simulink model "inverted_pendulum_simulink"  (R2025a)
settings: Solver=ode45  StartTime=0.0  StopTime=20  MaxStep=0.01  RelTol=1e-3
settings Model: Creator=user  LastModifiedBy=user

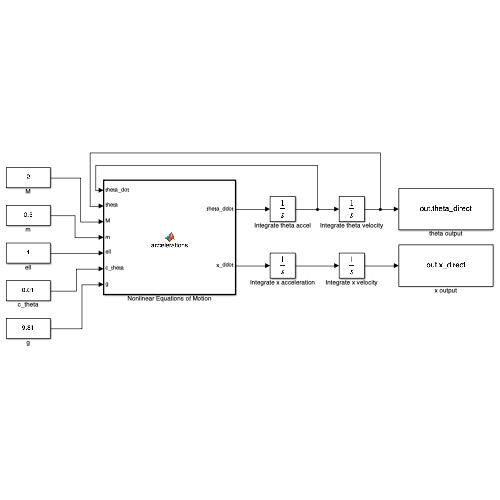
[thumbnail: Simulink's stored preview of the top-level diagram]
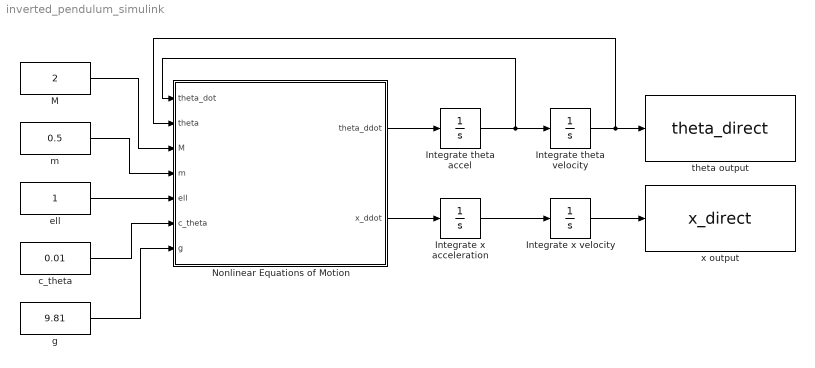
== system inverted_pendulum_simulink ==
  Integrate theta accel : Integrator
  Integrate theta velocity : Integrator  InitialCondition=0.087266462599716474
  Integrate x acceleration : Integrator
  Integrate x velocity : Integrator
  M : Constant  Value=2
  Nonlinear Equations of Motion : MATLAB Function  TreatAsAtomicUnit=on
  c_theta : Constant  Value=0.01
  ell : Constant
  g : Constant  Value=9.81
  m : Constant  Value=0.5
  theta output : ToWorkspace  VariableName=theta_direct  SaveFormat=Timeseries  SampleTime=-1
  x output : ToWorkspace  VariableName=x_direct  SaveFormat=Timeseries  SampleTime=-1
  wires:
  Integrate x acceleration/1 -> Integrate x velocity/1
  Integrate x velocity/1 -> x output/1
  Integrate theta accel/1 -> Integrate theta velocity/1, Nonlinear Equations of Motion/1(theta_dot)
  Integrate theta velocity/1 -> theta output/1, Nonlinear Equations of Motion/2(theta)
  M/1 -> Nonlinear Equations of Motion/3(M)
  m/1 -> Nonlinear Equations of Motion/4(m)
  ell/1 -> Nonlinear Equations of Motion/5(ell)
  c_theta/1 -> Nonlinear Equations of Motion/6(c_theta)
  g/1 -> Nonlinear Equations of Motion/7(g)
  Nonlinear Equations of Motion/1(theta_ddot) -> Integrate theta accel/1
  Nonlinear Equations of Motion/2(x_ddot) -> Integrate x acceleration/1

== matlab function inverted_pendulum_simulink/Nonlinear Equations of Motion ==
  data: theta_dot input; theta_ddot output; theta input; x_ddot output; M input; m input; ell input; c_theta input; g input
function [theta_ddot, x_ddot] = accelerations(theta_dot, theta, M, m, ell, c_theta, g)
% Solve the coupled nonlinear mass-matrix equations.
s = sin(theta);
c = cos(theta);
mass_matrix = [M + m, m * ell * c; m * ell * c, m * ell^2];
forcing = [m * ell * s * theta_dot^2; m * g * ell * s - c_theta * theta_dot];
acceleration = mass_matrix \ forcing;
x_ddot = acceleration(1);
theta_ddot = acceleration(2);
end
